simulink subsystem "laplaceStopConditionComputation"  (R2024b)
settings: Solver=VariableStepAuto  StartTime=0.0  StopTime=10.0  RelTol=1e-3
undefined symbols (not defined in the file): environment
settings Model: Creator=pierb  LastModifiedBy=pierb

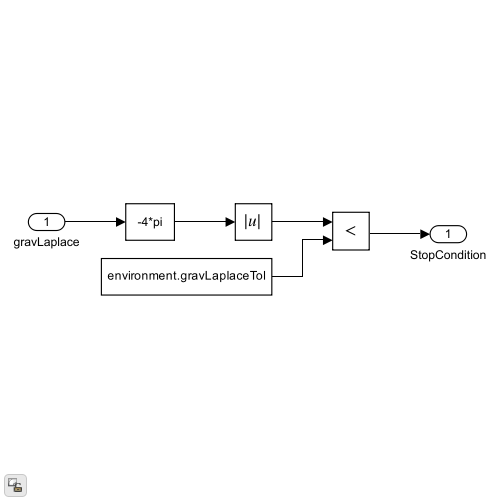
[thumbnail: Simulink's stored preview of the top-level diagram]
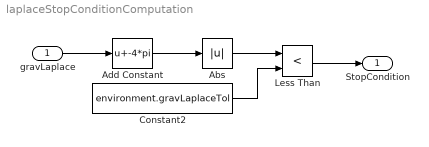
== system laplaceStopConditionComputation ==
  gravLaplace : Inport
  Abs : Abs  SaturateOnIntegerOverflow=off
  Add Constant : Bias  Bias=-4*pi  SaturateOnIntegerOverflow=off
  Constant2 : Constant  Value=environment.gravLaplaceTol
  Less Than : RelationalOperator  Operator=<  OutDataTypeStr=boolean  RndMeth=Simplest  InputSameDT=off
  StopCondition : Outport
  wires:
  Constant2/1 -> Less Than/2
  gravLaplace/1 -> Add Constant/1
  Abs/1 -> Less Than/1
  Add Constant/1 -> Abs/1
  Less Than/1 -> StopCondition/1
